simulink model "prueba_1_adcTors232"  (Simulink 7.1)
settings: Solver=FixedStepDiscrete  StartTime=0.0  StopTime=10.0  FixedStep=0.001  RelTol=1e-3
undefined symbols (not defined in the file or in its folder): Aceleraciones, DiscIntNeverNeededParam, u1, u2, u3, y1
libraries: dsPICdrivers x5, simulink x4
settings Model: Creator=Cesar  LastModifiedBy=Cesar
settings OptimizationCC: OptimizeModelRefInitCode=on  LifeSpan=1
settings HardwareCC: ProdBitPerInt=16  ProdEndianess=LittleEndian  ProdWordSize=16  ProdHWDeviceType=16-bit Generic
settings RTWCC: SystemTargetFile=dspic.tlc  TemplateMakefile=dspic_pic30_gcc.tmf  PostCodeGenCommand=dsPIC_Compile()  Description=Embedded Target for Microchip dsPIC (real-time)  ProcessScript=dspic_make_rtw_hook
settings CodeAppCC: IgnoreCustomStorageClasses=off
settings STFCustomTargetCC: ModelReferenceCompliant=off  IncludeMdlTerminateFcn=off  CombineOutputUpdateFcns=on  SuppressErrorStatus=on  ERTCustomFileBanners=on  SupportContinuousTime=off  SupportNonInlinedSFcns=off  SystemTargetFile=dspic.tlc
settings ERTTargetCC: ModelReferenceCompliant=off  CompOptLevelCompliant=off  IncludeMdlTerminateFcn=off  SuppressErrorStatus=on  ERTFirstTimeCompliant=off  ModelStepFunctionPrototypeControlCompliant=off  InlinedParameterPlacement=NonHierarchical  ERTSrcFileBannerTemplate=dsPIC_code_template.cgt  ERTHdrFileBannerTemplate=dsPIC_code_template.cgt  ERTDataSrcFileTemplate=dsPIC_code_template.cgt  ERTDataHdrFileTemplate=dsPIC_code_template.cgt  ERTCustomFileTemplate=dsPIC_main.tlc
settings CustomProperty: DataType=string  Value=C:\PROGRA~1\MATLAB\R2008a\bin\win32\gmake

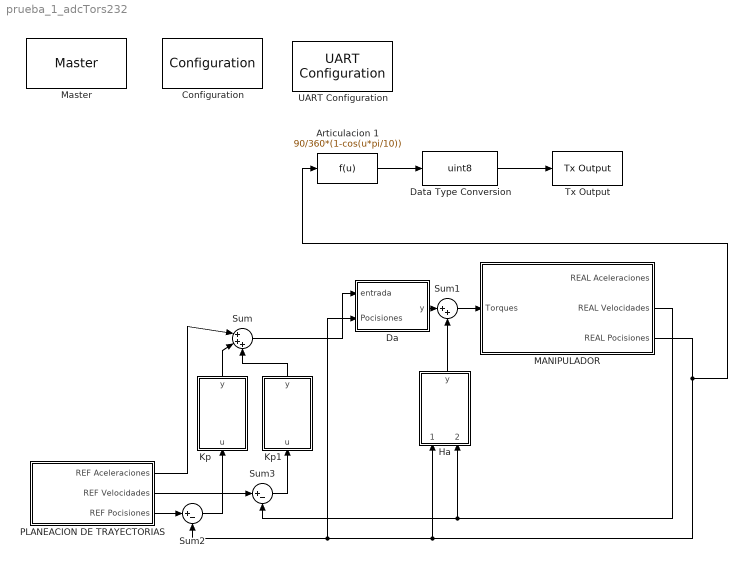
== system prueba_1_adcTors232 ==
  Articulacion 1 : Fcn  Expr=90/360*(1-cos(u*pi/10))  SampleTime=0.001
  Configuration : dsPICdrivers/Configuration  SystemSampleTime=-1  double64=on
  Da : Stateflow chart
  Data Type Conversion : DataTypeConversion  OutDataTypeMode=uint8  OutDataType=sfix(16)  OutScaling=2^0  OutDataTypeStr=uint8
  Ha : Stateflow chart  Orientation=up
  Kp : Stateflow chart  Orientation=up
  Kp1 : Stateflow chart  Orientation=up
  MANIPULADOR : Subsystem
  Master : dsPICdrivers/Master  Tag=dsPIC_MASTER  Priority=1  TimeStepType=Timer1  picType=30f4011  fcy=5e6  Quartz_33f=5e6  PLLActive_33f=off  fcyDesired_33f=0  tmr1="[1  4999  0]"  tmr1Info="Time Step : 0.001  ;   Error : 0%  PR1=4999"  tmr2345="[0  0  0  0]"  tmr2345cfg=[-1 -1 -1 -1]  IOautoConf=on  typePort="[ 0  0  0  0  0  0  0  0  0  0  0  0  0  0  0  0  0  0  0  0  0  0  0  0  0  0  0  0  0  0  0  0  0  0  0  0  0  0  0  0  0  0  0  0  0  5  4  0  0  0  0  0  0  0  0  0  0  0  0  0  0  0  0  0  0  0  0  0  0  0  0  0  0  0  0  0  0  0  0  0  0  0  0  0  0  0  0  0  0  0  0  0  0  0  0  0  0  0  0  0  0  0  0  0  0  0  0  0  0  0  0  0 ]"  TRIS="[ 65535  65535  65535  65535  65535  65535  65535 ]"  ADPCFG=0  MasterBusyPort=None  MasterOverloadPort=None  FOSC=LP  TempProtection_33f=TEMP_ON  FPBOR=PBOR_OFF  PWRT=PWRT_OFF  MCLR=MCLR_EN  PowerSave=off
  PLANEACION DE TRAYECTORIAS : Subsystem
  Sum : Sum  Inputs=|+++  OutDataType=sfix(16)  OutScaling=2^0
  Sum1 : Sum  Inputs=|++  OutDataType=sfix(16)  OutScaling=2^0
  Sum2 : Sum  Inputs=|+-  OutDataType=sfix(16)  OutScaling=2^0
  Sum3 : Sum  Inputs=|+-  OutDataType=sfix(16)  OutScaling=2^0
  Tx Output : dsPICdrivers/Serial PORT/Tx Output  Tag=dsPIC_TX  Priority=5  UART=1  OrderingInOutPopup=None
  UART Configuration : dsPICdrivers/Serial PORT/UART Configuration  Tag=dsPIC_config_UART  Priority=2  UART=1  proposed_BAUD=9600  ALT_TX_RX=on  InterruptTxWhen=When Transmit Buffer is empty  TXInterruptPri=1  TxBufferSize=32  TXEN=on  InterruptRxWhen=When Receive Buffer is full (contain 4 characters)  RXInterruptPri=2  RxBufferSize=32  BAUD=9600  UxBRG=32  Info="UxBRG = 32   ||  Real Baud : 9470   ||  % error : -1.3573  ||  max 0.94697 Bytes / Step"  RealBaud=0
  wires:
  Data Type Conversion/1 -> Tx Output/1
  Articulacion 1/1 -> Data Type Conversion/1
  Sum2/1 -> Kp/1(u)
  MANIPULADOR/3(REAL Pocisiones) -> Sum2/2, Da/2(Pocisiones), Ha/1(Pocisiones), Articulacion 1/1
  PLANEACION DE TRAYECTORIAS/2(REF Velocidades) -> Sum3/1
  MANIPULADOR/2(REAL Velocidades) -> Sum3/2, Ha/2(Velocidades)
  Kp/1(y) -> Sum/2
  Sum3/1 -> Kp1/1(u)
  Kp1/1(y) -> Sum/3
  PLANEACION DE TRAYECTORIAS/1(REF Aceleraciones) -> Sum/1
  Sum/1 -> Da/1(entrada)
  Sum1/1 -> MANIPULADOR/1(Torques)
  Ha/1(y) -> Sum1/2
  Da/1(y) -> Sum1/1
  PLANEACION DE TRAYECTORIAS/3(REF Pocisiones) -> Sum2/1

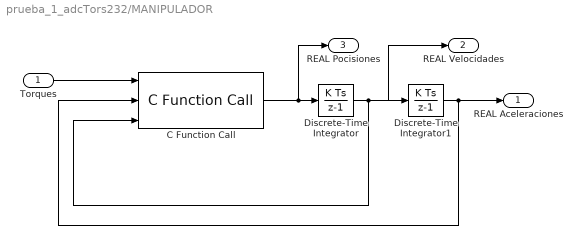
== system prueba_1_adcTors232/MANIPULADOR ==
  Torques : Inport  OutDataType=sfix(16)  OutScaling=2^0
  C Function Call : dsPICdrivers/OTHERS/C Function Call  Tag=dsPIC_dsPIC_CFunctionCall  fctName='Aceleraciones'  INPUT_SIZE=2  INPUT1=uint32  INPUT2=uint32  INPUT3=uint32  OUTPUT_SIZE=2  OUTPUT1=uint32  SampleTime=0.001  InputType=[ 6 6 6 ]  OutputType=[ 6 ]  FctDeclaration=extern void Aceleraciones(uint32_T* u1, uint32_T* u2, uint32_T* u3,uint32_T* y1);  FctCall=Aceleraciones(*%u1, *%u2, *%u3, *%y1);  OrderingInOutPopup=None
  Discrete-Time Integrator : DiscreteIntegrator  SampleTime=0.001  OutDataTypeMode=uint32  OutDataType=sfix(16)  OutScaling=2^0  OutDataTypeStr=uint32  ICPrevOutput=DiscIntNeverNeededParam  ICPrevScaledInput=DiscIntNeverNeededParam
  Discrete-Time Integrator1 : DiscreteIntegrator  SampleTime=0.001  OutDataTypeMode=uint32  OutDataType=sfix(16)  OutScaling=2^0  OutDataTypeStr=uint32  ICPrevOutput=DiscIntNeverNeededParam  ICPrevScaledInput=DiscIntNeverNeededParam
  REAL Aceleraciones : Outport  OutDataType=sfix(16)  OutScaling=2^0
  REAL Velocidades : Outport  Port=2  OutDataType=sfix(16)  OutScaling=2^0
  REAL Pocisiones : Outport  Port=3  OutDataType=sfix(16)  OutScaling=2^0
  wires:
  C Function Call/1 -> REAL Pocisiones/1, Discrete-Time Integrator/1
  Torques/1 -> C Function Call/1
  Discrete-Time Integrator/1 -> REAL Velocidades/1, Discrete-Time Integrator1/1, C Function Call/3
  Discrete-Time Integrator1/1 -> REAL Aceleraciones/1, C Function Call/2

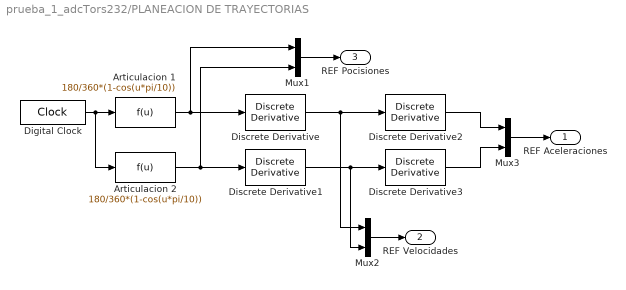
== system prueba_1_adcTors232/PLANEACION DE TRAYECTORIAS ==
  Articulacion 1 : Fcn  Expr=180/360*(1-cos(u*pi/10))  SampleTime=0.001
  Articulacion 2 : Fcn  Expr=180/360*(1-cos(u*pi/10))  SampleTime=0.001
  Digital Clock : DigitalClock  SampleTime=0.001
  Discrete Derivative{,1..3} (4 alike) : simulink/Discrete/Discrete Derivative  SystemSampleTime=-1  gainval=1.0  ICPrevScaledInput=0.0  OutMin=[]  OutMax=[]  OutDataType=sfix(16)  OutScaling=2^-10  DoSatur=off
  Mux1 : Mux  Inputs=2
  Mux2 : Mux  Inputs=2
  Mux3 : Mux  Inputs=2
  REF Aceleraciones : Outport  OutDataType=sfix(16)  OutScaling=2^0
  REF Velocidades : Outport  Port=2  OutDataType=sfix(16)  OutScaling=2^0
  REF Pocisiones : Outport  Port=3  OutDataType=sfix(16)  OutScaling=2^0
  wires:
  Digital Clock/1 -> Articulacion 1/1, Articulacion 2/1
  Mux3/1 -> REF Aceleraciones/1
  Mux2/1 -> REF Velocidades/1
  Mux1/1 -> REF Pocisiones/1
  Articulacion 1/1 -> Mux1/1, Discrete Derivative/1
  Articulacion 2/1 -> Mux1/2, Discrete Derivative1/1
  Discrete Derivative/1 -> Mux2/1, Discrete Derivative2/1
  Discrete Derivative1/1 -> Mux2/2, Discrete Derivative3/1
  Discrete Derivative2/1 -> Mux3/1
  Discrete Derivative3/1 -> Mux3/2

== matlab function Kp ==
  data: u input double size=2; y output double size=2
function y = Kp(u)
% This block supports an embeddable subset of the MATLAB language.
% See the help menu for details. 

y = [1000,0;0,1000]*u;

== matlab function Kp1 ==
  data: u input double size=2; y output double size=2
function y = Kv(u)
% This block supports an embeddable subset of the MATLAB language.
% See the help menu for details. 

y = [100,0;0,100]*u;

== matlab function Da ==
  data: entrada input double size=2; y output double size=2; Pocisiones input double size=2
function y = Da(entrada,Pocisiones)
% This block supports an embeddable subset of the MATLAB language.
% See the help menu for details. 
P_thet2=Pocisiones(2,1);
D=[.123e8*cos(P_thet2)+.121e9, .613e7*cos(P_thet2)+.974e7;.613e7*cos(P_thet2)+.974e7,.974e7];
y =D*entrada;

== matlab function Ha ==
  data: Pocisiones input double size=2; y output double size=2; Velocidades input double
function y = ha(Pocisiones,Velocidades)
% This block supports an embeddable subset of the MATLAB language.
% See the help menu for details. 

P_thet1=Pocisiones(1,1);
P_thet2=Pocisiones(2,1);
V_thet1=Velocidades(1,1);
V_thet2=Velocidades(2,1);

H=[ -.613e7*V_thet2*sin(P_thet2)*(2.*V_thet1+V_thet2);.613e7*V_thet1^2*sin(P_thet2)];
y = H;
